simulink model "w6_stage4_3_avg"  (R2026a)
settings: Solver=ode23t  StopTime=2  MaxStep=2.5e-05  RelTol=1e-6  AbsTol=1e-9
libraries: sm_lib x4, nesl_utility x4
settings Model: Creator=cogml  LastModifiedBy=cogml
settings SimscapeCC: SimscapeLogType=none
settings ExplorerConfigSet: SimMechanicsOpenEditorOnUpdate=off

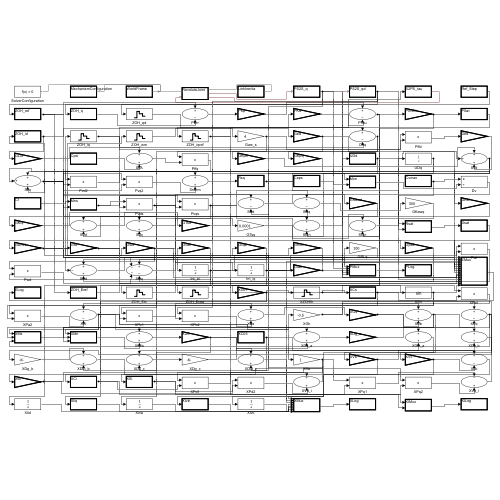
[thumbnail: Simulink's stored preview of the top-level diagram]
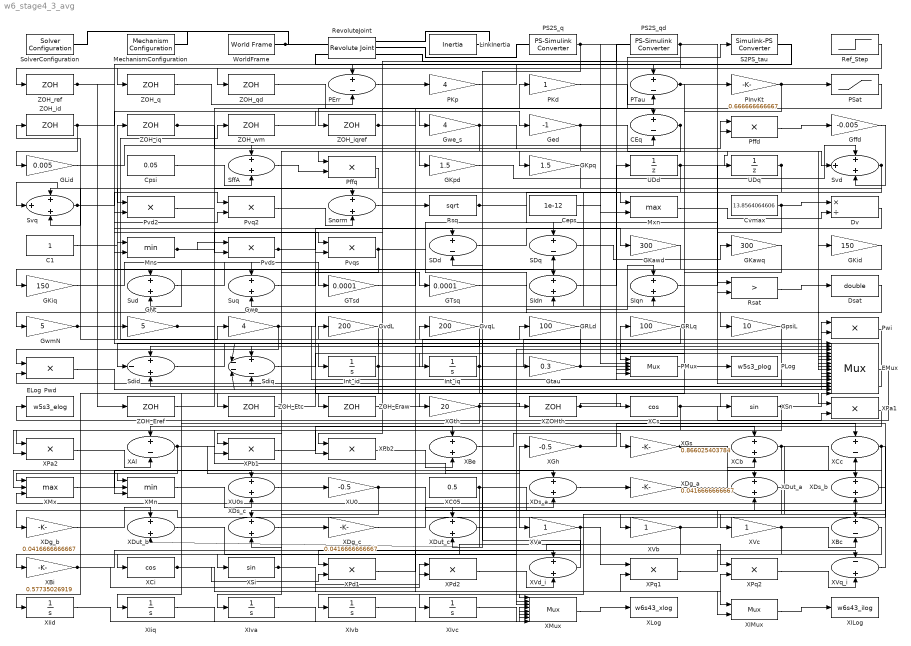
== system w6_stage4_3_avg ==
  C1 : Constant
  CEq : Sum  Inputs=+-
  Ceps : Constant  Value=1e-12
  Cpsi : Constant  Value=0.05
  Cvmax : Constant  Value=13.8564064606
  Dsat : DataTypeConversion  OutDataTypeStr=double  SaturateOnIntegerOverflow=off  RndMeth=Floor
  Dv : Product  Inputs=*/
  ELog : ToWorkspace  VariableName=w5s3_elog  SaveFormat=Timeseries  SampleTime=0.0001
  EMux : Mux  Inputs=16
  GKawd : Gain  Gain=300
  GKawq : Gain  Gain=300
  GKid : Gain  Gain=150
  GKiq : Gain  Gain=150
  GKpd : Gain  Gain=1.5
  GKpq : Gain  Gain=1.5
  GLid : Gain  Gain=0.005
  GNt : Gain  Gain=5
  GRLd : Gain  Gain=100
  GRLq : Gain  Gain=100
  GTsd : Gain  Gain=0.0001
  GTsq : Gain  Gain=0.0001
  Ged : Gain  Gain=-1
  Gffd : Gain  Gain=-0.005
  GpsiL : Gain  Gain=10
  Gtau : Gain  Gain=0.3
  GvdL : Gain  Gain=200
  GvqL : Gain  Gain=200
  Gwe : Gain  Gain=4
  Gwe_s : Gain  Gain=4
  GwmN : Gain  Gain=5
  Int_id : Integrator
  Int_iq : Integrator
  LinkInertia : sm_lib/Body Elements/Inertia  InertiaType=Custom  Mass=1  MassUnits=kg  CenterOfMass=[0.2 0 0]  CenterOfMassUnits=m  MomentsOfInertia=[0.000416666666667 0.0135416666667 0.0160416666667]  MomentsOfInertiaUnits=kg*m^2  ProductsOfInertia=[0 0 0]  ProductsOfInertiaUnits=kg*m^2  GraphicType=Marker  MarkerShape=Inertia  MarkerSize=20  GraphicVisPropType=SimpleVisualProperties  GraphicDiffuseColor=[0.5 0.5 0.5]  GraphicOpacity=1  GraphicSpecularColor=[0.5 0.5 0.5 1.0]  GraphicAmbientColor=[0.15 0.15 0.15 1.0]  GraphicEmissiveColor=[0.0 0.0 0.0 1.0]  GraphicShininess=75
  MechanismConfiguration : sm_lib/Utilities/Mechanism Configuration  UniformGravity=None  GravityVector=[0 0 -9.80665]  GravityVectorUnits=m/s^2  LinearizationDelta=0.001  JointModeTransitionNonlinearIterations=2
  Mns : MinMax  Inputs=2
  Mxn : MinMax  Function=max  Inputs=2
  PErr : Sum  Inputs=+-
  PInvKt : Gain  Gain=0.666666666667
  PKd : Gain
  PKp : Gain  Gain=4
  PLog : ToWorkspace  VariableName=w5s3_plog  SaveFormat=Timeseries  SampleTime=0.001
  PMux : Mux  Inputs=5
  PS2S_q : nesl_utility/PS-Simulink Converter  PhysicalDomain=network_engine_domain  SubClassName=ps_output  LeftPortType=input  RightPortType=output  PseudoPeriodic=off  Frequencies=[]  VectorFormat=inherit  Unit=rad  AffineConversion=off
  PS2S_qd : nesl_utility/PS-Simulink Converter  PhysicalDomain=network_engine_domain  SubClassName=ps_output  LeftPortType=input  RightPortType=output  PseudoPeriodic=off  Frequencies=[]  VectorFormat=inherit  Unit=rad/s  AffineConversion=off
  PSat : Saturate  UpperLimit=2  LowerLimit=-2
  PTau : Sum  Inputs=+-
  Pffd : Product
  Pffq : Product
  Pvd2 : Product
  Pvds : Product
  Pvq2 : Product
  Pvqs : Product
  Pwd : Product
  Pwi : Product
  Ref_Step : Step  Time=0.1995  FinalValue=0.3  SampleTime=0
  RevoluteJoint : sm_lib/Joints/Revolute Joint  JointMode=Normal  CompositeWrenchDir=FollowerOnBase  CompositeWrenchFrame=BaseFrame  SenseConstraintForce=off  SenseConstraintTorque=off  SenseTotalForce=off  SenseTotalTorque=off  PositionTargetSpecify=off  PositionTargetPriority=High  PositionTargetValue=0  PositionTargetValueUnits=deg  VelocityTargetSpecify=off  VelocityTargetPriority=High  VelocityTargetValue=0  VelocityTargetValueUnits=deg/s  EquilibriumPosition=0  EquilibriumPositionUnits=deg  SpringStiffness=0  SpringStiffnessUnits=N*m/deg  DampingCoefficient=0.1  DampingCoefficientUnits=N*m/(rad/s)  LowerLimitSpecify=off  LowerLimitBound=-90  LowerLimitBoundUnits=deg  LowerLimitStiffness=1e4  LowerLimitStiffnessUnits=N*m/deg  LowerLimitDamping=10  LowerLimitDampingUnits=N*m/(deg/s)  LowerLimitTransitionRegionWidth=0.1  LowerLimitTransitionRegionWidthUnits=deg  UpperLimitSpecify=off  UpperLimitBound=90  UpperLimitBoundUnits=deg  UpperLimitStiffness=1e4  UpperLimitStiffnessUnits=N*m/deg  UpperLimitDamping=10  UpperLimitDampingUnits=N*m/(deg/s)  UpperLimitTransitionRegionWidth=0.1  UpperLimitTransitionRegionWidthUnits=deg  TorqueActuationMode=InputTorque  MotionActuationMode=ComputedMotion  SensePosition=on  SenseVelocity=on  SenseAcceleration=off  SenseTorqueForce=off  SenseLowerLimitTorqueForce=off  SenseUpperLimitTorqueForce=off
  Rsat : RelationalOperator  Operator=>  OutDataTypeStr=boolean  RndMeth=Simplest  InputSameDT=off
  Rsq : Sqrt
  S2PS_tau : nesl_utility/Simulink-PS Converter  PhysicalDomain=network_engine_domain  SubClassName=ps_input  LeftPortType=input  RightPortType=output  PseudoPeriodic=off  Frequencies=[]  NoiseDistribution=none  NoiseParameters=[]  Unit=N*m  AffineConversion=off  FilteringAndDerivatives=provide  SimscapeFilterOrder=1  InputFilterTimeConstant=0.001  UdotUserProvided=0
  SDd : Sum  Inputs=+-
  SDq : Sum  Inputs=+-
  SIdn : Sum
  SIqn : Sum
  Sdid : Sum  Inputs=+-+
  Sdiq : Sum  Inputs=+---
  SffA : Sum
  Snorm : Sum
  SolverConfiguration : nesl_utility/Solver Configuration  PhysicalDomain=network_engine_domain  SubClassName=solver  LeftPortType=input  RightPortType=generic  Tones=[]  Harmonics=[]  SimulateNoise=off  Profile=off  UseLocalSampling=off  EnableSwitchedLinearOptims=on  FrequencyDomain=off  UseCCode=off  RelTol=0.001  AbsTol=0.001  MinStep=1e-09  ToWorkspace=off  RevertToSquareIcSolve=off  NumHomotopyIterations=100  PhasorMode=off  PhasorModeNumHarmonics=1  ConsistencySolver=NEWTON_XTOL_AFTER_FTOL  CanonicalOrdering=CANONICAL  OptimizeIntermediates=OPTIMIZED  IndexReductionMethod=DerivativeReplacement  DoDC=off  ResidualTolerance=1e-09  ConsistencyTolSource=GLOBAL  ConsistencyAbsTol=0.001  ConsistencyRelTol=0.001  ConsistencyTolFactor=0.001  UseLocalSolver=off  LocalSolverChoice=NE_BACKWARD_EULER_ADVANCER  ResolveIndetEquations=on  FunctionEvalNumThread=1  LocalSolverSampleTime=0.001  DoFixedCost=off  MaxNonlinIter=3  MaxModeIter=2  ComputeImpulses=off  ImpulseIterations=2  LinearAlgebra=auto  LinearAlgebraNumThread=0  EquationFormulation=NE_TIME_EF  DelaysMemoryBudget=1024  AutomaticFiltering=on  FilteringTimeConstant=0.001  PartitionStorageMethod=AS_NEEDED  PartitionMemoryBudget=1024  PartitionMethod=ROBUST  MultibodyUseLocalSolver=off  MultibodyLocalSolverChoice=ODE1  MultibodyLocalSolverSampleTime=0.001
  Sud : Sum
  Suq : Sum
  Svd : Sum  Inputs=+++
  Svq : Sum  Inputs=+++
  UDd : UnitDelay  SampleTime=0.0001
  UDq : UnitDelay  SampleTime=0.0001
  WorldFrame : sm_lib/Frames and Transforms/World Frame
  XAl : Sum  Inputs=+-
  XBc : Sum  Inputs=+-
  XBe : Sum
  XBi : Gain  Gain=0.57735026919
  XC05 : Constant  Value=0.5
  XCb : Sum
  XCc : Sum  Inputs=+-
  XCi : Trigonometry  Operator=cos
  XCs : Trigonometry  Operator=cos
  XDg_a : Gain  Gain=0.0416666666667
  XDg_b : Gain  Gain=0.0416666666667
  XDg_c : Gain  Gain=0.0416666666667
  XDs_a : Sum
  XDs_b : Sum
  XDs_c : Sum
  XDut_a : Sum
  XDut_b : Sum
  XDut_c : Sum
  XGh : Gain  Gain=-0.5
  XGs : Gain  Gain=0.866025403784
  XGth : Gain  Gain=20
  XILog : ToWorkspace  VariableName=w6s43_ilog  SaveFormat=Timeseries  SampleTime=-1
  XIMux : Mux  Inputs=2
  XIid : Integrator
  XIiq : Integrator
  XIva : Integrator
  XIvb : Integrator
  XIvc : Integrator
  XLog : ToWorkspace  VariableName=w6s43_xlog  SaveFormat=Timeseries  SampleTime=0.0001
  XMn : MinMax  Inputs=3
  XMux : Mux  Inputs=8
  XMx : MinMax  Function=max  Inputs=3
  XPa1 : Product
  XPa2 : Product
  XPb1 : Product
  XPb2 : Product
  XPd1 : Product
  XPd2 : Product
  XPq1 : Product
  XPq2 : Product
  XSi : Trigonometry
  XSn : Trigonometry
  XU0 : Gain  Gain=-0.5
  XU0s : Sum
  XVa : Gain
  XVb : Gain
  XVc : Gain
  XVd_i : Sum
  XVq_i : Sum  Inputs=-+
  XZOHth : ZeroOrderHold  SampleTime=0.0001
  ZOH_Eraw : ZeroOrderHold  SampleTime=0.0001
  ZOH_Eref : ZeroOrderHold  SampleTime=0.0001
  ZOH_Etc : ZeroOrderHold  SampleTime=0.0001
  ZOH_id : ZeroOrderHold  SampleTime=0.0001
  ZOH_iq : ZeroOrderHold  SampleTime=0.0001
  ZOH_iqref : ZeroOrderHold  SampleTime=0.0001
  ZOH_q : ZeroOrderHold  SampleTime=0.001
  ZOH_qd : ZeroOrderHold  SampleTime=0.001
  ZOH_ref : ZeroOrderHold  SampleTime=0.001
  ZOH_wm : ZeroOrderHold  SampleTime=0.0001
  wires:
  Ref_Step/1 -> ZOH_ref/1
  PS2S_q/1 -> ZOH_q/1, PMux/2, EMux/12, XGth/1
  PS2S_qd/1 -> ZOH_qd/1, GwmN/1, PMux/3, EMux/13
  ZOH_ref/1 -> PErr/1, PMux/1, ZOH_Eref/1
  ZOH_q/1 -> PErr/2
  PErr/1 -> PKp/1
  ZOH_qd/1 -> PKd/1
  PKp/1 -> PTau/1
  PKd/1 -> PTau/2
  PTau/1 -> PInvKt/1, PMux/4, ZOH_Etc/1
  PInvKt/1 -> PSat/1, ZOH_Eraw/1
  GwmN/1 -> Gwe/1, ZOH_wm/1, EMux/9
  Pvds/1 -> SDd/1, EMux/6, XPa1/1, XPb1/1
  Pvqs/1 -> SDq/1, EMux/7, XPa2/1, XPb2/1
  Int_id/1 -> GRLd/1, Pwd/2, ZOH_id/1, EMux/2, XIid/1, XIMux/1
  Int_iq/1 -> GRLq/1, Pwi/2, Gtau/1, ZOH_iq/1, EMux/3, XIiq/1, XIMux/2
  Gwe/1 -> Pwi/1, Pwd/1, GpsiL/1
  GvdL/1 -> Sdid/1
  GRLd/1 -> Sdid/2
  Pwi/1 -> Sdid/3
  GvqL/1 -> Sdiq/1
  GRLq/1 -> Sdiq/2
  Pwd/1 -> Sdiq/3
  GpsiL/1 -> Sdiq/4
  Sdid/1 -> Int_id/1
  Sdiq/1 -> Int_iq/1
  PSat/1 -> ZOH_iqref/1
  ZOH_wm/1 -> Gwe_s/1
  ZOH_id/1 -> Ged/1, GLid/1
  ZOH_iqref/1 -> CEq/1, EMux/1
  ZOH_iq/1 -> CEq/2, Pffd/2
  Gwe_s/1 -> Pffd/1, Pffq/1
  Pffd/1 -> Gffd/1
  GLid/1 -> SffA/1
  Cpsi/1 -> SffA/2
  SffA/1 -> Pffq/2
  Ged/1 -> GKpd/1, GKid/1
  CEq/1 -> GKpq/1, GKiq/1
  GKpd/1 -> Svd/1
  UDd/1 -> Svd/2, SIdn/2
  Gffd/1 -> Svd/3
  GKpq/1 -> Svq/1
  UDq/1 -> Svq/2, SIqn/2
  Pffq/1 -> Svq/3
  Svd/1 -> Pvd2/1, Pvd2/2, Pvds/2, SDd/2, EMux/4
  Svq/1 -> Pvq2/1, Pvq2/2, Pvqs/2, SDq/2, EMux/5
  Pvd2/1 -> Snorm/1
  Pvq2/1 -> Snorm/2
  Snorm/1 -> Rsq/1
  Rsq/1 -> Mxn/1, Rsat/1
  Ceps/1 -> Mxn/2
  Cvmax/1 -> Dv/1, Rsat/2
  Mxn/1 -> Dv/2
  C1/1 -> Mns/1
  Dv/1 -> Mns/2
  Mns/1 -> Pvds/1, Pvqs/1
  SDd/1 -> GKawd/1
  SDq/1 -> GKawq/1
  GKid/1 -> Sud/1
  GKawd/1 -> Sud/2
  GKiq/1 -> Suq/1
  GKawq/1 -> Suq/2
  Sud/1 -> GTsd/1
  Suq/1 -> GTsq/1
  GTsd/1 -> SIdn/1
  SIdn/1 -> UDd/1
  GTsq/1 -> SIqn/1
  SIqn/1 -> UDq/1
  Rsat/1 -> Dsat/1
  Gtau/1 -> GNt/1, EMux/10
  GNt/1 -> S2PS_tau/1, PMux/5, EMux/15
  PMux/1 -> PLog/1
  Dsat/1 -> EMux/8
  ZOH_Eref/1 -> EMux/11
  ZOH_Etc/1 -> EMux/14
  ZOH_Eraw/1 -> EMux/16
  EMux/1 -> ELog/1
  XGth/1 -> XZOHth/1, XCi/1, XSi/1
  XZOHth/1 -> XCs/1, XSn/1
  XCs/1 -> XPa1/2, XPb2/2
  XSn/1 -> XPa2/2, XPb1/2
  XPa1/1 -> XAl/1
  XPa2/1 -> XAl/2
  XPb1/1 -> XBe/1
  XPb2/1 -> XBe/2
  XAl/1 -> XGh/1, XMx/1, XMn/1, XDs_a/1, XVa/1
  XBe/1 -> XGs/1
  XGh/1 -> XCb/1, XCc/1
  XGs/1 -> XCb/2, XCc/2
  XCb/1 -> XMx/2, XMn/2, XDs_b/1, XVb/1
  XCc/1 -> XMx/3, XMn/3, XDs_c/1, XVc/1
  XMx/1 -> XU0s/1
  XMn/1 -> XU0s/2
  XU0s/1 -> XU0/1
  XU0/1 -> XDs_a/2, XDs_b/2, XDs_c/2
  XDs_a/1 -> XDg_a/1
  XDg_a/1 -> XDut_a/1
  XC05/1 -> XDut_a/2, XDut_b/2, XDut_c/2
  XDs_b/1 -> XDg_b/1
  XDg_b/1 -> XDut_b/1
  XDs_c/1 -> XDg_c/1
  XDg_c/1 -> XDut_c/1
  XVb/1 -> XBc/1, XIvb/1
  XVc/1 -> XBc/2, XIvc/1
  XBc/1 -> XBi/1
  XVa/1 -> XPd1/1, XPq1/1, XIva/1
  XCi/1 -> XPd1/2, XPq2/2
  XBi/1 -> XPd2/1, XPq2/1
  XSi/1 -> XPd2/2, XPq1/2
  XPd1/1 -> XVd_i/1
  XPd2/1 -> XVd_i/2
  XPq1/1 -> XVq_i/1
  XPq2/1 -> XVq_i/2
  XVd_i/1 -> GvdL/1
  XVq_i/1 -> GvqL/1
  XDut_a/1 -> XMux/1
  XDut_b/1 -> XMux/2
  XDut_c/1 -> XMux/3
  XIid/1 -> XMux/4
  XIiq/1 -> XMux/5
  XIva/1 -> XMux/6
  XIvb/1 -> XMux/7
  XIvc/1 -> XMux/8
  XMux/1 -> XLog/1
  XIMux/1 -> XILog/1
  connections:
  RevoluteJoint/LConn1 -- WorldFrame/RConn1 -- SolverConfiguration/RConn1 -- MechanismConfiguration/RConn1
  RevoluteJoint/RConn1 -- LinkInertia/RConn1
  RevoluteJoint/RConn2 -- PS2S_q/LConn1
  RevoluteJoint/RConn3 -- PS2S_qd/LConn1
  S2PS_tau/RConn1 -- RevoluteJoint/LConn2
